simulink model "ACCable_Predefined_Inductance_Modelling_Study"  (R2024b)
settings: Solver=VariableStepAuto  StartTime=0.0  StopTime=10.0  RelTol=1e-3
libraries: ee_lib x3, fl_lib x1, nesl_utility x1
settings Model: Creator=SUDHAK1  LastModifiedBy=SUDHAK1

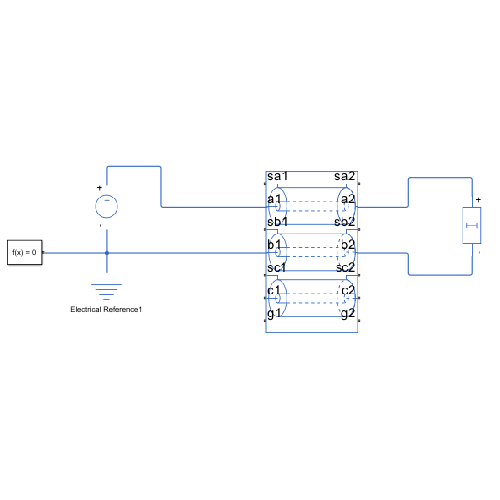
[thumbnail: Simulink's stored preview of the top-level diagram]
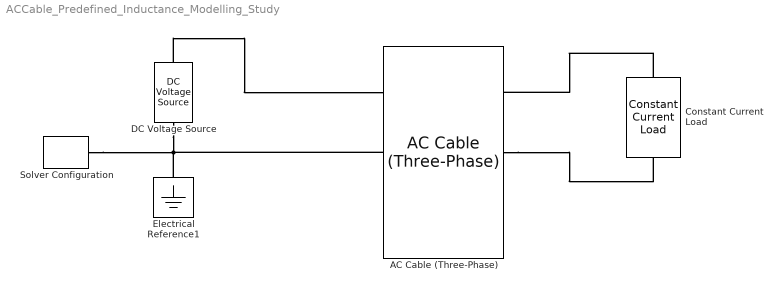
== system ACCable_Predefined_Inductance_Modelling_Study ==
  AC Cable (Three-Phase) : ee_lib/Passive/Lines/AC Cable (Three-Phase)  l=120 km  gmr=5 mm  srad=10 mm  cablerad=20 mm  Dab=25 mm  formation=1  Ra=1 Ohm/km  Rs=10 Ohm/km  epsr=2.4  epsr_env=1  prm=1  f=60 Hz  rho=100 Ohm*m  De=1 km  Rg=0.1 Ohm/km
      settings: InternalSimscapePortConfiguration="{\"Bottom\":[],\"Left\":[{\"id\":\"sa1\",\"label\":\"sa1\",\"type\":\"foundation.electrical.electrical\"},{\"id\":\"a1\",\"label\":\"a1\",\"type\":\"foundation.electrical.electrical\"},{\"id\":\"sb1\",\"label\":\"sb1\",\"type\":\"foundation.electrical.electrical\"},{\"id\":\"b1\",\"label\":\"b1\",\"type\":\"foundation.electrical.electrical\"},{\"id\":\"sc1\",\"label\":\"sc1\",\"type\":\"foundation.electrical.electrical\"},{\"id\":\"c1\",\"label\":\"c1\",\"type\":\"foundation.electrical.electrical\"},{\"id\":\"g1\",\"label\":\"g1\",\"type\":\"foundation.electrical.electrical\"}],\"Right\":[{\"id\":\"sa2\",\"label\":\"sa2\",\"type\":\"foundation.electrical.electrical\"},{\"id\":\"a2\",\"label\":\"a2\",\"type\":\"foundation.electrical.electrical\"},{\"id\":\"sb2\",\"label\":\"sb2\",\"type\":\"foundation.electrical.electrical\"},{\"id\":\"b2\",\"label\":\"b2\",\"type\":\"foundation.electrical.electrical\"},{\"id\":\"sc2\",\"label\":\"sc2\",\"type\":\"foundation.electrical.electrical\"},{\"id\":\"c2\",\"label\":\"c2\",\"type\":\"foundation.electrical.electrical\"},{\"id\":\"g2\",\"label\":\"g2\",\"type\":\"foundation.electrical.electrical\"}],\"Top\":[]}"
  Constant Current Load : ee_lib/Passive/Constant Current Load  load_type=ee.enum.dc_ac.dc  consumed_current=1 A  min_supply_voltage=5 V  G_reverse=1e-6 S  deltaV=1e-3 V  consumed_current_rms=100 A  f0=60 Hz  Vrms_min=200 V  fault_action=simscape.enum.assert.action.none  t_fault=1 s
      settings: InternalSimscapePortConfiguration="{\"Bottom\":[],\"Left\":[{\"id\":\"p\",\"label\":\"+\",\"type\":\"foundation.electrical.electrical\"}],\"Right\":[{\"id\":\"n\",\"label\":\"-\",\"type\":\"foundation.electrical.electrical\"}],\"Top\":[]}"
  DC Voltage Source : ee_lib/Additional Components/SPICE Sources/DC Voltage Source  DC=0 V
  Electrical Reference1 : fl_lib/Electrical/Electrical Elements/Electrical Reference
  Solver Configuration : nesl_utility/Solver Configuration  PhysicalDomain=network_engine_domain  SubClassName=solver  LeftPortType=input  RightPortType=generic  Tones=[]  Harmonics=[]  SimulateNoise=off  Profile=off  UseLocalSampling=off  EnableSwitchedLinearOptims=on  FrequencyDomain=off  UseCCode=off  RelTol=0.001  AbsTol=0.001  MinStep=1e-09  ToWorkspace=off  RevertToSquareIcSolve=off  NumHomotopyIterations=100  PhasorMode=off  PhasorModeNumHarmonics=1  ConsistencySolver=NEWTON_XTOL_AFTER_FTOL  IndexReductionMethod=DerivativeReplacement  DoDC=off  ResidualTolerance=1e-09  ConsistencyTolSource=GLOBAL  ConsistencyAbsTol=0.001  ConsistencyRelTol=0.001  ConsistencyTolFactor=0.001  UseLocalSolver=off  LocalSolverChoice=NE_BACKWARD_EULER_ADVANCER  ResolveIndetEquations=on  FunctionEvalNumThread=1  LocalSolverSampleTime=0.001  DoFixedCost=off  MaxNonlinIter=3  MaxModeIter=2  ComputeImpulses=off  ImpulseIterations=2  LinearAlgebra=auto  LinearAlgebraNumThread=0  EquationFormulation=NE_TIME_EF  DelaysMemoryBudget=1024  AutomaticFiltering=on  FilteringTimeConstant=0.001  PartitionStorageMethod=AS_NEEDED  PartitionMemoryBudget=1024  PartitionMethod=ROBUST  MultibodyUseLocalSolver=off  MultibodyLocalSolverChoice=ODE1  MultibodyLocalSolverSampleTime=0.001
  connections:
  Solver Configuration/RConn1 -- AC Cable (Three-Phase)/LConn4 -- Electrical Reference1/LConn1 -- DC Voltage Source/RConn1
  AC Cable (Three-Phase)/RConn4 -- Constant Current Load/RConn1
  Constant Current Load/LConn1 -- AC Cable (Three-Phase)/RConn2
  DC Voltage Source/LConn1 -- AC Cable (Three-Phase)/LConn2
